simulink model "Lab3_Task_3_a"  (R2025b)
settings: Solver=FixedStepAuto  StartTime=0.0  StopTime=inf  MaxStep=0.1  RelTol=1e-3  EnableMultiTasking=on
PreLoadFcn:
  | % load parameters of the default quadrotor
  | disp('Quadrotor parameters loaded by PreLoadFcn')
  | mdl_quadrotor
undefined symbols (not defined in the file or in its folder): Angular, Linear, rot2
libraries: robotlib x3
settings Model: Creator=corkep  LastModifiedBy=abodynasser22
settings SolverCC: AlgebraicLoopSolver=TrustRegion
settings DataIOCC: LimitDataPoints=on  ReturnWorkspaceOutputs=off
settings OptimizationCC: DefaultParameterBehavior=Inlined  EnhancedBackFolding=on  PassReuseOutputArgsAs=Individual arguments  ExpressionDepthLimit=2147483647.0  ZeroExternalMemoryAtStartup=off  ZeroInternalMemoryAtStartup=off  MaxStackSize=64  OptimizeBlockOrder=speed  DifferentSizesBufferReuse=on  OptimizationCustomize=off  EfficientTunableParamExpr=on
settings DebuggingCC: UnderspecifiedInitializationDetection=Classic  MergeDetectMultiDrivingBlocksExec=none  SolverPrmCheckMsg=warning  ParameterTunabilityLossMsg=error  UnconnectedInputMsg=warning  UnconnectedOutputMsg=warning  UnconnectedLineMsg=warning  AllowSymbolicDim=off  StateNameClashWarn=warning  SFUnexpectedBacktrackingDiag=warning  SFNoUnconditionalDefaultTransitionDiag=warning  SFExecutionAtInitializationDiag=none  ArithmeticOperatorsInVariantConditions=warning
settings HardwareCC: ProdBitPerLong=64.0  ProdHWDeviceType=Intel->x86-64 (Linux 64)  UseEmbeddedCoderFeatures=off
settings ModelReferenceCC: EnableRefExpFcnMdlSchedulingChecks=on  PropagateSignalLabelsOutOfModel=off
settings SFSimCC: SimUseLocalCustomCode=off  MATLABDynamicMemAlloc=off  CustomCodeUndefinedFunction=UseInterfaceOnly
settings RTWCC: SystemTargetFile=ert.tlc  HardwareBoard=Robot Operating System 2 (ROS 2)  TLCOptions="-aInlineSetEventsForThisBaseRateFcn=TLC_FALSE -aSuppressMultiTaskScheduler=TLC_FALSE  -aRateBasedStepFcn=0"  TemplateMakefile=ert_default_tmf  RTWUseLocalCustomCode=off  Toolchain=Colcon Tools  TargetLang=C++  GPUComputeCapability=3.5  DLArmComputeVersion=19.05  Description=Embedded Coder
settings CodeAppCC: ForceParamTrailComments=on  IgnoreCustomStorageClasses=off  OperatorAnnotations=on  SimulinkDataObjDesc=on  SFDataObjDesc=on  InsertBlockDesc=on
settings ERTTargetCC: ExtModeTransport=2.0  ExtModeStaticAlloc=on  ExtModeMexFile=ext_xcp  ExtModeIntrfLevel=Level2 - Open  RootIOFormat=Structure reference  CodeInterfacePackaging=C++ class  SupportNonInlinedSFcns=on
settings ConfigComp: CovMetricSettings=dw  CovSaveCumulativeToWorkspaceVar=on  CovSaveSingleToWorkspaceVar=on  CovExternalEMLEnable=off  CovSFcnEnable=off

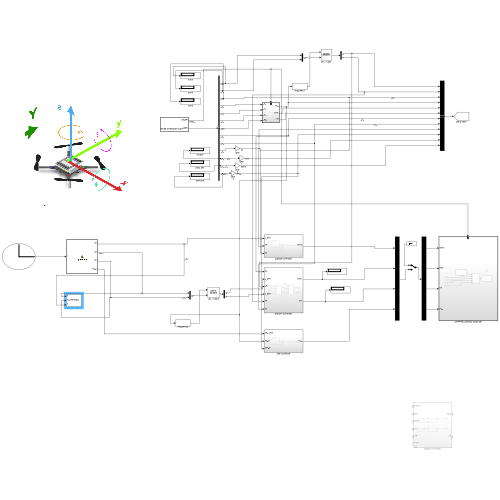
[thumbnail: Simulink's stored preview of the top-level diagram]
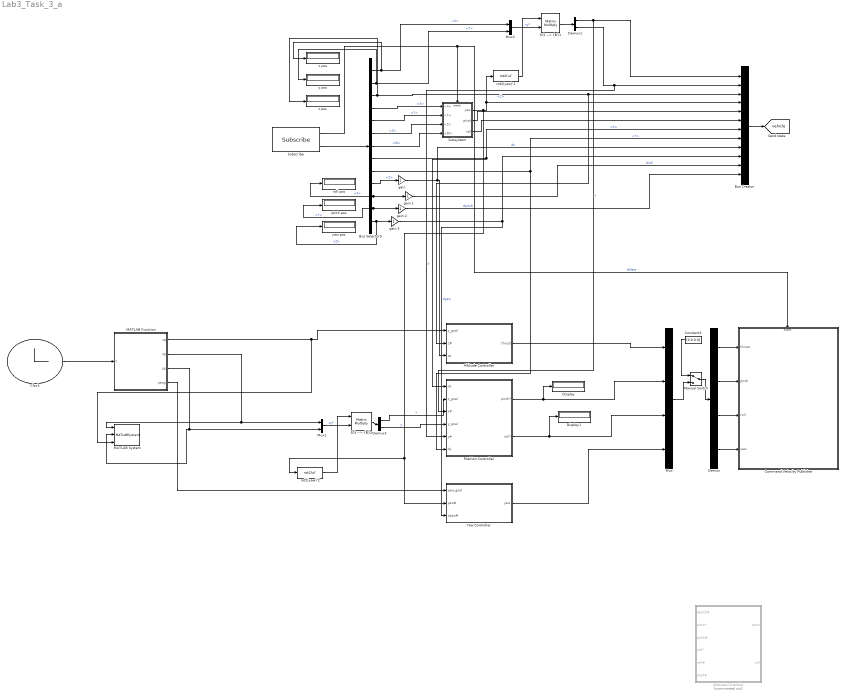
== system Lab3_Task_3_a ==
  Altitude Controller : Subsystem
  Attitude Controller : Subsystem  Commented=on
  Bus Creator : BusCreator  Inputs=12
  Bus Selector3 : BusSelector  OutputSignals=Pose.Pose.Position.X,Pose.Pose.Position.Y,Pose.Pose.Position.Z,Pose.Pose.Orientation.X,Pose.Pose.Orientation.Y,Pose.Pose.Orientation.Z,Pose.Pose.Orientation.W,Twist.Twist.Linear.X,Twist.Twist.Linear.Y,Twist.Twist.Linear.Z,Twist.Twist.Angular.X,Twist.Twist.Angular.Y,Twist.Twist.Angular.Z
  Clock : Clock
  Command Velocity Publisher : Subsystem
  Constant3 : Constant  Value=[0 0 0 0]
  Demux : Demux
  Demux1 : Demux  Outputs=2
  Demux3 : Demux  Outputs=2
  Display : Display
  Display1 : Display
  MATLAB Function : MATLAB Function  TreatAsAtomicUnit=on
  MATLAB System : MATLABSystem  System=LivePlot3D  SimulateUsing=Interpreted execution
      mask Type: LivePlot3D
  Manual Switch : ManualSwitch
  Mux : Mux
  Mux1 : Mux  Inputs=2
  Mux2 : Mux  Inputs=2
  Position Controller : Subsystem
  Subscribe : robotlib/Subscribe  topicSource=Select from ROS network  topic=/pixy/vicon/crazyflie1/crazyflie1/odom  messageType=nav_msgs/Odometry  SampleTime=-1  legacyBusStruct=off  messageQueueLength=51
  Subsystem : Subsystem
  Yaw Controller : Subsystem
  gain {,1..3} (4 alike) : Gain
  pitch pos : Display
  roll pos : Display
  rot2(yaw)'1 : MATLABFcn  MATLABFcn=rot2(u)'  OutputDimensions=[2 2]  Output1D=off
  rot2(yaw)'2 : MATLABFcn  MATLABFcn=rot2(u)'  OutputDimensions=[2 2]  Output1D=off
  x pos : Display
  y pos : Display
  yaw pos : Display
  z pos : Display
  "{0} --> {B}1" : Product  Multiplication=Matrix(*)  RndMeth=Zero
  "{0} --> {B}2" : Product  Multiplication=Matrix(*)  RndMeth=Zero
  tag scope: vehicle=global
  wires:
  Bus Selector3/11 -> gain 1/1, roll pos/1  "<X>"
  Bus Selector3/13 -> yaw pos/1, gain 3/1  "<Z>"
  Bus Selector3/10 -> "gain "/1  "<Z>"
  Bus Selector3/9 -> Position Controller/6(dy), Bus Creator/8  "<Y>"
  Bus Selector3/8 -> Bus Creator/7, Position Controller/1(dx)  "<X>"
  Bus Selector3/3 -> z pos/1, Altitude Controller/2(z#), Bus Creator/3  "<Z>"
  Bus Creator/1 -> [vehicle]
  Bus Selector3/12 -> gain 2/1, pitch pos/1  "<Y>"
  Subscribe/2 -> Bus Selector3/1
  Subscribe/1 -> Subsystem/Enable, Command Velocity Publisher/Enable  "IsNew"
  Mux2/1 -> "{0} --> {B}1"/2  "xy*"
  "{0} --> {B}1"/1 -> Demux1/1
  Demux1/1 -> Position Controller/3(x#), Bus Creator/1  "x"
  Demux1/2 -> Position Controller/5(y#), Bus Creator/2  "y"
  Bus Selector3/1 -> x pos/1, Mux2/1  "<X>"
  Bus Selector3/2 -> Mux2/2, y pos/1  "<Y>"
  rot2(yaw)'1/1 -> "{0} --> {B}1"/1
  "gain "/1 -> Altitude Controller/3(dz), Bus Creator/9  "dz"
  gain 1/1 -> Bus Creator/11  "droll"
  gain 2/1 -> Bus Creator/12  "dpitch"
  gain 3/1 -> Yaw Controller/3(dyaw#), Bus Creator/10  "dyaw"
  Subsystem/1(yaw) -> Yaw Controller/2(yaw#), rot2(yaw)'2/1, rot2(yaw)'1/1, Bus Creator/4
  Bus Selector3/4 -> Subsystem/1(<X>)  "<X>"
  Bus Selector3/5 -> Subsystem/2(<Y>)  "<Y>"
  Bus Selector3/6 -> Subsystem/3(<Z>)  "<Z>"
  Bus Selector3/7 -> Subsystem/4(<W>)  "<W>"
  Subsystem/2(pitch) -> Bus Creator/5
  Subsystem/3(roll) -> Bus Creator/6
  Altitude Controller/1(thrust) -> Mux/1
  Constant3/1 -> Manual Switch/1
  Manual Switch/1 -> Demux/1
  Mux/1 -> Manual Switch/2
  Demux/1 -> Command Velocity Publisher/1(thrust)
  Demux/4 -> Command Velocity Publisher/4(yaw)
  Demux/2 -> Command Velocity Publisher/2(pitch)
  Demux/3 -> Command Velocity Publisher/3(roll)
  Position Controller/1(pitch*) -> Display/1, Mux/2
  Position Controller/2(roll*) -> Display1/1, Mux/3
  Yaw Controller/1(yaw) -> Mux/4
  "{0} --> {B}2"/1 -> Demux3/1
  rot2(yaw)'2/1 -> "{0} --> {B}2"/1
  Mux1/1 -> "{0} --> {B}2"/2  "xy*"
  Demux3/1 -> Position Controller/2(x_goal)  "x"
  Demux3/2 -> Position Controller/4(y_goal)  "y"
  MATLAB Function/2(xg) -> Mux1/1, MATLAB System/1
  MATLAB Function/4(yawg) -> Yaw Controller/1(yaw_goal)
  MATLAB Function/3(yg) -> Mux1/2, MATLAB System/2
  MATLAB Function/1(zg) -> MATLAB System/3, Altitude Controller/1(z_goal)
  Clock/1 -> MATLAB Function/1(t)

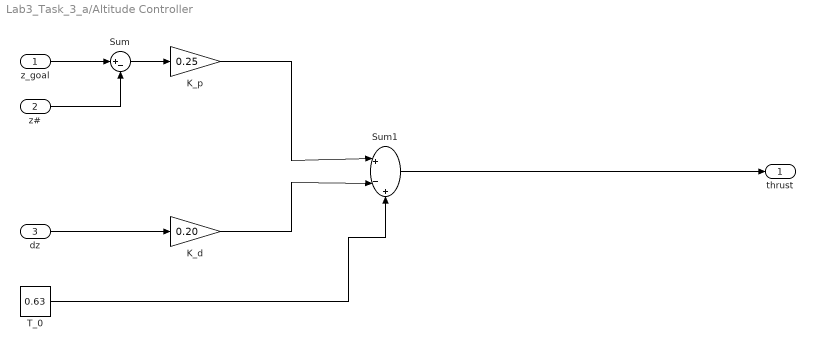
== system Lab3_Task_3_a/Altitude Controller ==
  z_goal : Inport  PortDimensions=1
  z# : Inport  Port=2
  dz : Inport  Port=3
  K_d : Gain  Gain=0.20
  K_p : Gain  Gain=0.25
  Sum : Sum  Inputs=|+-
  Sum1 : Sum  Inputs=|+-+
  T_0 : Constant  Value=0.63
  thrust : Outport
  wires:
  K_p/1 -> Sum1/1
  z#/1 -> Sum/2
  T_0/1 -> Sum1/3
  Sum/1 -> K_p/1
  z_goal/1 -> Sum/1
  K_d/1 -> Sum1/2
  Sum1/1 -> thrust/1
  dz/1 -> K_d/1

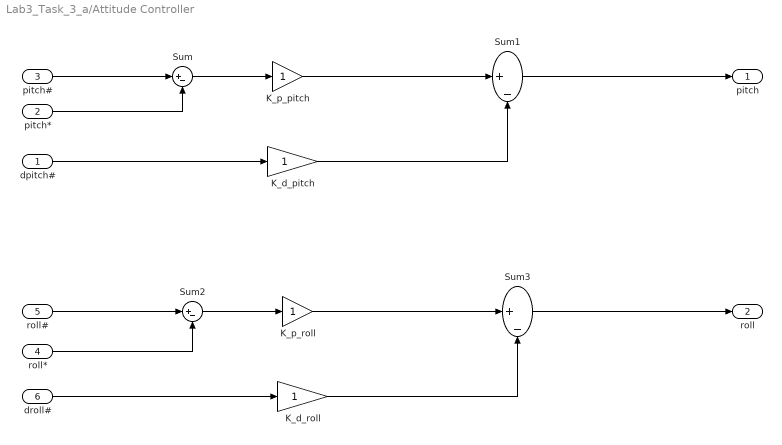
== system Lab3_Task_3_a/Attitude Controller ==
  dpitch# : Inport
  pitch* : Inport  Port=2
  pitch# : Inport  Port=3
  roll* : Inport  Port=4
  roll# : Inport  Port=5
  droll# : Inport  Port=6
  K_d_pitch : Gain
  K_d_roll : Gain
  K_p_pitch : Gain
  K_p_roll : Gain
  Sum{,1..3} (4 alike) : Sum  Inputs=|+-
  pitch : Outport
  roll : Outport  Port=2
  wires:
  Sum1/1 -> pitch/1
  pitch#/1 -> Sum/1
  K_p_pitch/1 -> Sum1/1
  dpitch#/1 -> K_d_pitch/1
  Sum/1 -> K_p_pitch/1
  K_d_pitch/1 -> Sum1/2
  pitch*/1 -> Sum/2
  K_p_roll/1 -> Sum3/1
  Sum2/1 -> K_p_roll/1
  K_d_roll/1 -> Sum3/2
  roll#/1 -> Sum2/1
  droll#/1 -> K_d_roll/1
  Sum3/1 -> roll/1
  roll*/1 -> Sum2/2

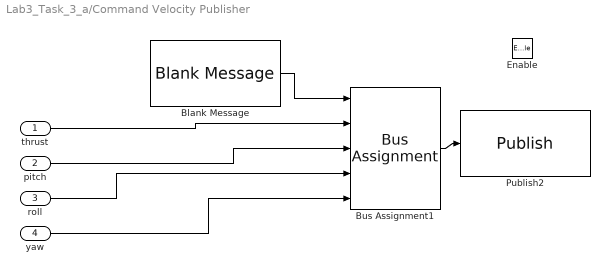
== system Lab3_Task_3_a/Command Velocity Publisher ==
  thrust : Inport
  pitch : Inport  Port=2
  roll : Inport  Port=3
  yaw : Inport  Port=4
  Enable : EnablePort
  Blank Message : robotlib/Blank Message  messageClass=Message  entityType=geometry_msgs/Twist  messageType=geometry_msgs/Twist  SampleTime=inf  legacyBusStruct=off
  Bus Assignment1 : BusAssignment  DialogController=Simulink.DDGSource_BusAssignment  AssignedSignals=Linear.Z,Linear.X,Linear.Y,Angular.Z
  Publish2 : robotlib/Publish  topicSource=Select from ROS network  topic=/crazyflie1/cmd_vel  messageType=geometry_msgs/Twist  legacyBusStruct=off  messageQueueLength=105
  wires:
  Bus Assignment1/1 -> Publish2/1
  Blank Message/1 -> Bus Assignment1/1
  yaw/1 -> Bus Assignment1/5
  roll/1 -> Bus Assignment1/4
  pitch/1 -> Bus Assignment1/3
  thrust/1 -> Bus Assignment1/2

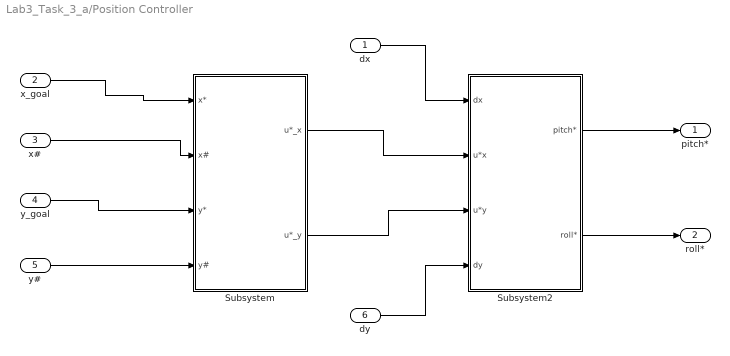
== system Lab3_Task_3_a/Position Controller ==
  dx : Inport
  x_goal : Inport  Port=2
  x# : Inport  Port=3
  y_goal : Inport  Port=4
  y# : Inport  Port=5
  dy : Inport  Port=6
  Subsystem : Subsystem
  Subsystem2 : Subsystem
  pitch* : Outport
  roll* : Outport  Port=2
  wires:
  x_goal/1 -> Subsystem/1(x*)
  y_goal/1 -> Subsystem/3(y*)
  y#/1 -> Subsystem/4(y#)
  x#/1 -> Subsystem/2(x#)
  Subsystem/1(u*_x) -> Subsystem2/2(u*x)
  Subsystem/2(u*_y) -> Subsystem2/3(u*y)
  dy/1 -> Subsystem2/4(dy)
  dx/1 -> Subsystem2/1(dx)
  Subsystem2/1(pitch*) -> pitch*/1
  Subsystem2/2(roll*) -> roll*/1

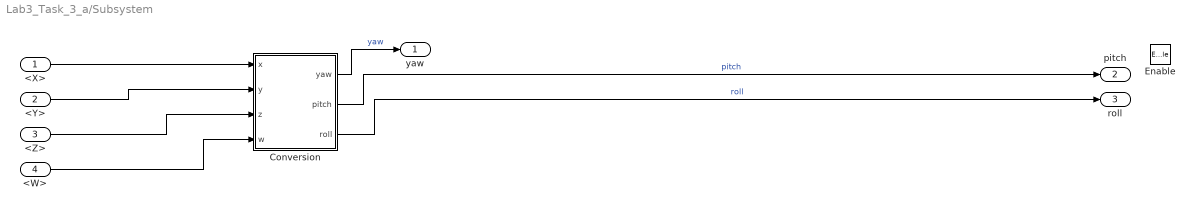
== system Lab3_Task_3_a/Subsystem ==
  <X> : Inport
  <Y> : Inport  Port=2
  <Z> : Inport  Port=3
  <W> : Inport  Port=4
  Enable : EnablePort
  Conversion : MATLAB Function  TreatAsAtomicUnit=on
  yaw : Outport
  pitch : Outport  Port=2
  roll : Outport  Port=3
  wires:
  Conversion/1(yaw) -> yaw/1  "yaw"
  <X>/1 -> Conversion/1(x)
  Conversion/2(pitch) -> pitch/1  "pitch"
  <W>/1 -> Conversion/4(w)
  <Y>/1 -> Conversion/2(y)
  Conversion/3(roll) -> roll/1  "roll"
  <Z>/1 -> Conversion/3(z)

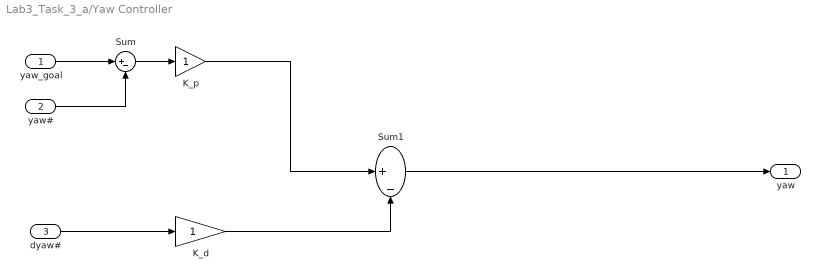
== system Lab3_Task_3_a/Yaw Controller ==
  yaw_goal : Inport  PortDimensions=1
  yaw# : Inport  Port=2
  dyaw# : Inport  Port=3
  K_d : Gain
  K_p : Gain
  Sum : Sum  Inputs=|+-
  Sum1 : Sum  Inputs=|+-
  yaw : Outport
  wires:
  K_p/1 -> Sum1/1
  yaw#/1 -> Sum/2
  Sum/1 -> K_p/1
  K_d/1 -> Sum1/2
  Sum1/1 -> yaw/1
  dyaw#/1 -> K_d/1
  yaw_goal/1 -> Sum/1

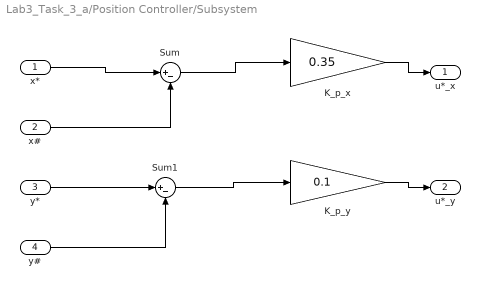
== system Lab3_Task_3_a/Position Controller/Subsystem ==
  x* : Inport
  x# : Inport  Port=2
  y* : Inport  Port=3
  y# : Inport  Port=4
  K_p_x : Gain  Gain=0.35
  K_p_y : Gain  Gain=0.1
  Sum : Sum  Inputs=|+-
  Sum1 : Sum  Inputs=|+-
  u*_x : Outport
  u*_y : Outport  Port=2
  wires:
  x*/1 -> Sum/1
  x#/1 -> Sum/2
  y*/1 -> Sum1/1
  y#/1 -> Sum1/2
  Sum/1 -> K_p_x/1
  Sum1/1 -> K_p_y/1
  K_p_y/1 -> u*_y/1
  K_p_x/1 -> u*_x/1

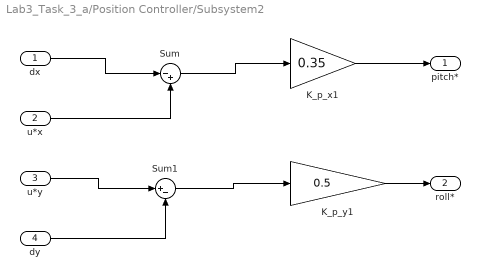
== system Lab3_Task_3_a/Position Controller/Subsystem2 ==
  dx : Inport
  u*x : Inport  Port=2
  u*y : Inport  Port=3
  dy : Inport  Port=4
  K_p_x1 : Gain  Gain=0.35
  K_p_y1 : Gain  Gain=0.5
  Sum : Sum  Inputs=|-+
  Sum1 : Sum  Inputs=|+-
  pitch* : Outport
  roll* : Outport  Port=2
  wires:
  dx/1 -> Sum/1
  u*x/1 -> Sum/2
  u*y/1 -> Sum1/1
  dy/1 -> Sum1/2
  Sum/1 -> K_p_x1/1
  Sum1/1 -> K_p_y1/1
  K_p_y1/1 -> roll*/1
  K_p_x1/1 -> pitch*/1

== matlab function Lab3_Task_3_a/Subsystem/Conversion ==
  data: yaw output; x input; y input; z input; w input; pitch output; roll output
function [yaw,pitch,roll]  = quat2eul(x,y,z,w)
%#codegen

% Convert the quaternion to a yaw angle (zyx euler angle)
eul = quat2eul([w,x,y,z]);
yaw = eul(1);
roll = eul(3);
pitch = eul(2);

end

== matlab function Lab3_Task_3_a/MATLAB Function ==
  data: t input; zg output; xg output; yg output; yawg output
function [zg, xg, yg, yawg] = square_traj_mstraj(t)
% Trajektoria för kvadrat med 2 s stopp i hörnen, baserad på mstraj.
% t  : aktuell tid (skalar)
% xg, yg, zg, yawg : referenser i ENA (världen)

    persistent tVec posRef yawRef z0 Ttot

    if isempty(tVec)
        %% --- Parametrar ---
        L     = 0.7;     % sidlängd [m]
        z0    = 1.0;     % konstant höjd
        v     = 0.2;     % hastighet på varje sida [m/s]
        Tedge = L / v;   % tid att flyga en sida
        Thold = 2.0;     % hålltid i hörn [s]
        dt    = 0.01;    % samplingssteg för referensen
        tacc  = 0.2;     % accelerationstid för mstraj (kan justeras)

        %% --- Hörn (ENA) ---
        P1 = [2   2];
        P2 = [L   2];
        P3 = [L   L];
        P4 = [2   L];

        % via-punkter för kvadrat + stopp i hörn
        P = [P2; P2; ...   % P1->P2 (flyg), P2->P2 (håll)
             P3; P3; ...   % P2->P3, håll i P3
             P4; P4; ...   % P3->P4, håll i P4
             P1; P1];      % P4->P1, håll i P1

        % segmenttider: flyg, håll, flyg, håll, ...
        Tseg = [Tedge Thold Tedge Thold Tedge Thold Tedge Thold];

        % --- Generera multi-segment-bana (bara x,y) ---
        % P: 8x2, start i P1
        posRef = mstraj(P, [], Tseg, P1, dt, tacc);   % Nx2

        % tidsvektor för en hel loop
        N    = size(posRef,1);
        tVec = (0:N-1)' * dt;
        Ttot = tVec(end);

        %% --- Yaw: titta mot nästa hörn ---
        yawRef = zeros(N,1);

        % riktningar sida 1–4
        yaw12 = atan2(P2(2)-P1(2), P2(1)-P1(1));  % P1->P2
        yaw23 = atan2(P3(2)-P2(2), P3(1)-P2(1));  % P2->P3
        yaw34 = atan2(P4(2)-P3(2), P4(1)-P3(1));  % P3->P4
        yaw41 = atan2(P1(2)-P4(2), P1(1)-P4(1));  % P4->P1

        nSeg  = round(Tseg / dt);
        kEnd  = cumsum(nSeg);

        % 1: flyg P1->P2, yaw mot P2
        yawRef(1:kEnd(1)) = yaw12;
        % 2: håll i P2, titta mot P3
        yawRef(kEnd(1)+1:kEnd(2)) = yaw23;
        % 3: flyg P2->P3, yaw mot P3
        yawRef(kEnd(2)+1:kEnd(3)) = yaw23;
        % 4: håll i P3, titta mot P4
        yawRef(kEnd(3)+1:kEnd(4)) = yaw34;
        % 5: flyg P3->P4
        yawRef(kEnd(4)+1:kEnd(5)) = yaw34;
        % 6: håll i P4, titta mot P1
        yawRef(kEnd(5)+1:kEnd(6)) = yaw41;
        % 7: flyg P4->P1
        yawRef(kEnd(6)+1:kEnd(7)) = yaw41;
        % 8: håll i P1, titta mot P2
        yawRef(kEnd(7)+1:kEnd(8)) = yaw12;
    end

    %% --- Slå upp referens för aktuell tid t ---
    % gör banan periodisk
    tau = mod(t, Ttot);

    % hitta närmaste tidindex
    [~, k] = min(abs(tVec - tau));

    xg   = posRef(k,1);
    yg   = posRef(k,2);
    zg   = z0;
    yawg = yawRef(k);
end
